simulink model "usv_heading_pid_model"  (R2024b)
settings: Solver=ode4  StartTime=0  StopTime=170  FixedStep=0.01  RelTol=1e-3
libraries: slpidlib x1
settings Model: Creator=qianr  LastModifiedBy=qianr
settings DataIOCC: SaveOutput=off

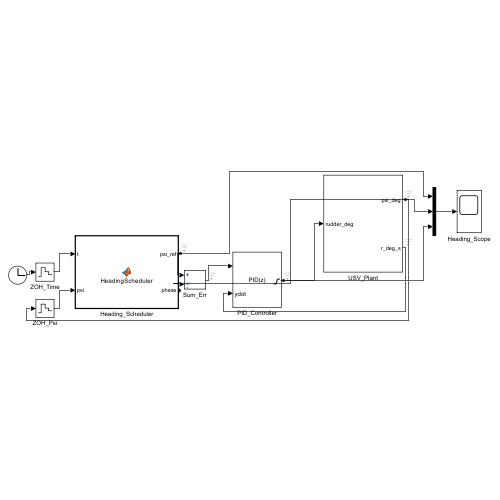
[thumbnail: Simulink's stored preview of the top-level diagram]
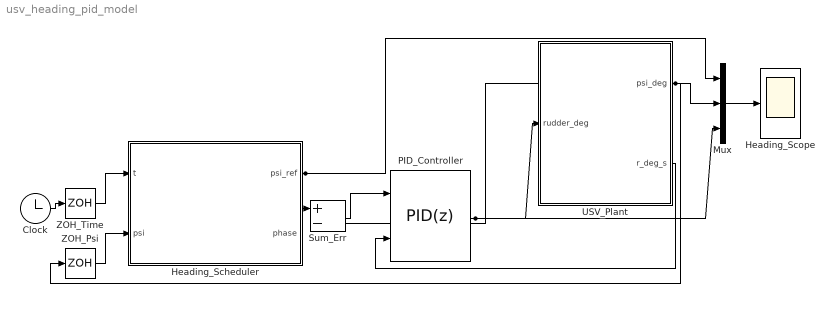
== system usv_heading_pid_model ==
  Clock : Clock
  Heading_Scheduler : MATLAB Function  TreatAsAtomicUnit=on
  Heading_Scope : Scope
  Mux : Mux  Inputs=3
  PID_Controller : slpidlib/PID Controller  Controller=PID  Form=Parallel  TimeDomain=Discrete-time  UseExternalTs=off  SampleTime=0.05  IntegratorMethod=Forward Euler  FilterMethod=Forward Euler  ControllerParametersSource=internal  P=7.56  I=1.08  UseKiTs=off  D=16.5  UseExternalDerivativeSource=on  N=20  UseFilter=on  TunerSelectOption=Transfer Function Based (PID Tuner App)  InitialConditionSource=internal  InitialConditionForIntegrator=0  InitialConditionForFilter=0  DifferentiatorICPrevScaledInput=0  ExternalReset=none  TrackingMode=off  Kt=1  LimitOutput=on  SatLimitsSource=internal  UpperSaturationLimit=30  LowerSaturationLimit=-30  LinearizeAsGain=on  AntiWindupMode=clamping  Kb=1  LimitIntegrator=off  UpperIntegratorSaturationLimit=inf  LowerIntegratorSaturationLimit=-inf  POutMin=[]  POutMax=[]  IOutMin=[]  IOutMax=[]  DOutMin=[]  DOutMax=[]  NOutMin=[]  NOutMax=[]  SumOutMin=[]  SumOutMax=[]  SaturationOutMin=[]  SaturationOutMax=[]  PParamMin=[]  PParamMax=[]  IParamMin=[]  IParamMax=[]  DParamMin=[]  DParamMax=[]  NParamMin=[]  NParamMax=[]  KbParamMin=[]  KbParamMax=[]  KtParamMin=[]  KtParamMax=[]  KbOutMin=[]  KbOutMax=[]  KtOutMin=[]  KtOutMax=[]  IntegratorOutMin=[]  IntegratorOutMax=[]  FilterOutMin=[]  FilterOutMax=[]  SumI1OutMin=[]  SumI1OutMax=[]  SumI2OutMin=[]  SumI2OutMax=[]  SumI3OutMin=[]  SumI3OutMax=[]  SumI4OutMin=[]  SumI4OutMax=[]  SumDOutMin=[]  SumDOutMax=[]  DifferentiatorOutMin=[]  DifferentiatorOutMax=[]  FilterDiffOutCoefMin=[]  FilterDiffOutCoefMax=[]  ReciprocalOutMin=[]  ReciprocalOutMax=[]  SumDenOutMin=[]  SumDenOutMax=[]  SumNumOutMin=[]  SumNumOutMax=[]  DivideOutMin=[]  DivideOutMax=[]  UdiffTsProdOutMin=[]  UdiffTsProdOutMax=[]  NTsProdOutMin=[]  NTsProdOutMax=[]  UintegralTsProdOutMin=[]  UintegralTsProdOutMax=[]  UngainTsProdOutMin=[]  UngainTsProdOutMax=[]  ClampingZeroOutDataTypeStr=Inherit: Inherit via back propagation  ClampingZeroOutMin=[]  ClampingZeroOutMax=[]  FilterDenConstantOutDataTypeStr=Inherit: Inherit via back propagation  FilterDenConstantOutMin=[]  FilterDenConstantOutMax=[]  PCopyOutDataTypeStr=Inherit: Inherit via back propagation  PCopyOutMin=[]  PCopyOutMax=[]  NCopyOutDataTypeStr=Inherit: Inherit via back propagation  NCopyOutMin=[]  NCopyOutMax=[]  IntegratorContinuousStateAttributes=''  IntegratorStateMustResolveToSignalObject=off  IntegratorRTWStateStorageClass=Auto  FilterContinuousStateAttributes=''  FilterStateMustResolveToSignalObject=off  FilterRTWStateStorageClass=Auto  ParallelPVariant=InternalParameters  IdealPVariant=Disabled  IVariant=InternalParameters  DVariant=InternalParameters  IntegratorVariant=Discrete  SatVariant=Enabled  AWVariant=DiscClampingParallel  PCopyVariant=Disabled  TRVariant=Disabled  FdbkBlocksVariant=Forward  IdealPFdbkVariant=Disabled  SatFdbkVariant=Disabled  DerivativeFilterVariant=ForwardEulerFilterOnly  NVariant=InternalParameters  NCopyVariant=Disabled  FilterICVariant=InternalICsFilter  IntegratorICVariant=InternalICs  ExternalResetVariant=Disabled  TRSumVariant=Passthrough  SumFdbkVariant=Disabled  SumVariant=Sum_PID  TsampFilterVariant=InternalTs  TsampNgainVariant=Passthrough  TsampIntegralVariant=Disabled_SignalSpec  ExternalSaturationOutDataTypeStr=Inherit: Same as second input  DerivativeSourceVariant=ExternalYdot  PreIntVariant=InternalPreInt
  Sum_Err : Sum  Inputs=+-
  USV_Plant : Subsystem
  ZOH_Psi : ZeroOrderHold  SampleTime=0.05
  ZOH_Time : ZeroOrderHold  SampleTime=0.05
  wires:
  Clock/1 -> ZOH_Time/1
  ZOH_Time/1 -> Heading_Scheduler/1(t)
  Heading_Scheduler/1(psi_ref) -> Sum_Err/1, Mux/1
  USV_Plant/1(psi_deg) -> Sum_Err/2, ZOH_Psi/1, Mux/2
  ZOH_Psi/1 -> Heading_Scheduler/2(psi)
  Sum_Err/1 -> PID_Controller/1
  USV_Plant/2(r_deg_s) -> PID_Controller/2
  PID_Controller/1 -> USV_Plant/1(rudder_deg), Mux/3
  Mux/1 -> Heading_Scope/1

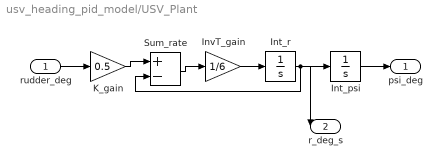
== system usv_heading_pid_model/USV_Plant ==
  rudder_deg : Inport
  Int_psi : Integrator
  Int_r : Integrator
  InvT_gain : Gain  Gain=1/6
  K_gain : Gain  Gain=0.5
  Sum_rate : Sum  Inputs=+-
  psi_deg : Outport
  r_deg_s : Outport  Port=2
  wires:
  rudder_deg/1 -> K_gain/1
  K_gain/1 -> Sum_rate/1
  Sum_rate/1 -> InvT_gain/1
  InvT_gain/1 -> Int_r/1
  Int_r/1 -> Int_psi/1, Sum_rate/2, r_deg_s/1
  Int_psi/1 -> psi_deg/1

== matlab function usv_heading_pid_model/Heading_Scheduler ==
  data: t input; psi_ref output; psi input; phase output
function [psi_ref, phase] = HeadingScheduler(t, psi)
%#codegen
% Heading command scheduler with a +-0.1 deg / 10 s dwell criterion.
persistent ph tHold
if isempty(ph)
    ph = 1;
    tHold = -1;
end
targets = [30, 230, 30];
tol = 0.1;
holdReq = 10;
if abs(psi - targets(ph)) < tol
    if tHold < 0
        tHold = t;
    end
    if (t - tHold) >= holdReq && ph < 3
        ph = ph + 1;
        tHold = -1;
    end
else
    tHold = -1;
end
psi_ref = targets(ph);
phase = ph;
